simulink model "untitled"  (R2019a)
settings: Solver=ode4  StartTime=0.0  StopTime=100  FixedStep=0.0001  RelTol=1e-3
settings Model: Creator=bahaa  LastModifiedBy=bahaa

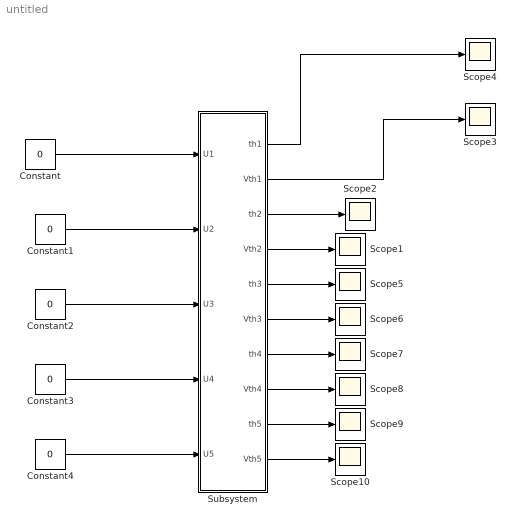
== system untitled ==
  Constant{,1..4} (5 alike) : Constant  Value=0
  Scope{1..10} (10 alike) : Scope
  Subsystem : Subsystem
  wires:
  Constant1/1 -> Subsystem/2(U2)
  Subsystem/4(Vth2) -> Scope1/1
  Constant/1 -> Subsystem/1(U1)
  Constant2/1 -> Subsystem/3(U3)
  Constant3/1 -> Subsystem/4(U4)
  Constant4/1 -> Subsystem/5(U5)
  Subsystem/3(th2) -> Scope2/1
  Subsystem/2(Vth1) -> Scope3/1
  Subsystem/1(th1) -> Scope4/1
  Subsystem/5(th3) -> Scope5/1
  Subsystem/6(Vth3) -> Scope6/1
  Subsystem/7(th4) -> Scope7/1
  Subsystem/8(Vth4) -> Scope8/1
  Subsystem/9(th5) -> Scope9/1
  Subsystem/10(Vth5) -> Scope10/1

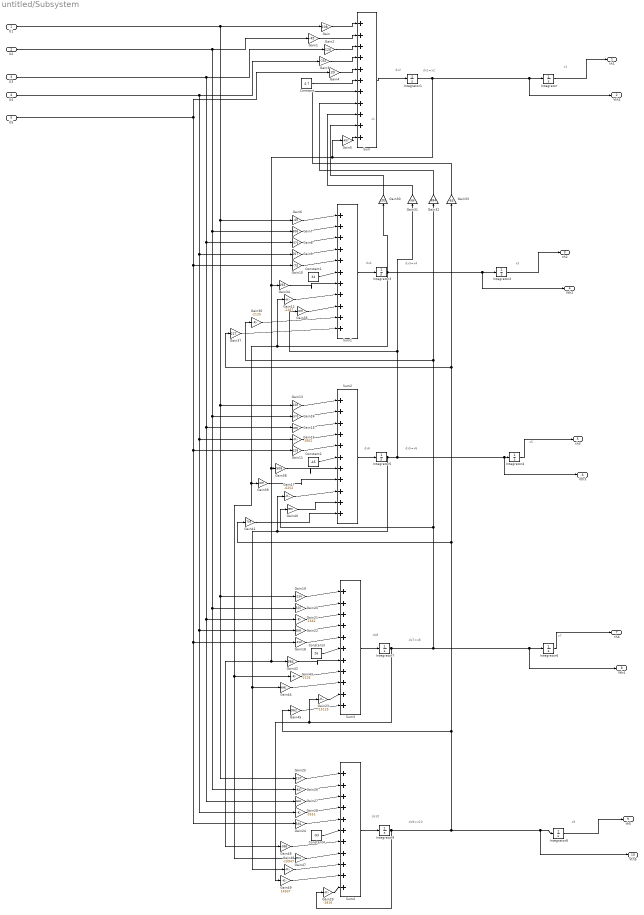
== system untitled/Subsystem ==
  note: dx1=x2
  note: x1
  note: dx2
  note: x3
  note: dx3=x4
  note: x1
  note: x5
  note: dx5=x6
  note: dx7=x8
  note: x7
  note: dx9=x10
  note: x9
  note: dx4
  note: dx6
  note: dx8
  note: dx10
  U1 : Inport
  U2 : Inport  Port=2
  U3 : Inport  Port=3
  U4 : Inport  Port=4
  U5 : Inport  Port=5
  Constant : Constant  Value=4.7
  Constant1 : Constant  Value=34
  Constant2 : Constant  Value=-45
  Constant3 : Constant  Value=26
  Constant4 : Constant  Value=-93
  Gain : Gain  Gain=108
  Gain1 : Gain  Gain=-45
  Gain10 : Gain  Gain=-73
  Gain11 : Gain  Gain=229
  Gain12 : Gain  Gain=-1287
  Gain13 : Gain  Gain=120
  Gain14 : Gain  Gain=-570
  Gain15 : Gain  Gain=1486
  Gain16 : Gain  Gain=-1662
  Gain17 : Gain  Gain=-6252
  Gain18 : Gain  Gain=-313
  Gain19 : Gain  Gain=-234
  Gain2 : Gain  Gain=120
  Gain20 : Gain  Gain=507
  Gain21 : Gain  Gain=-1662
  Gain22 : Gain  Gain=3595
  Gain23 : Gain  Gain=-15125
  Gain24 : Gain  Gain=591
  Gain25 : Gain  Gain=237
  Gain26 : Gain  Gain=-837
  Gain27 : Gain  Gain=2602
  Gain28 : Gain  Gain=-3551
  Gain29 : Gain  Gain=-1816
  Gain3 : Gain  Gain=-234
  Gain30 : Gain  Gain=192
  Gain31 : Gain  Gain=-506
  Gain32 : Gain  Gain=984
  Gain33 : Gain  Gain=-64
  Gain34 : Gain  Gain=192
  Gain35 : Gain  Gain=2400
  Gain36 : Gain  Gain=-2135
  Gain37 : Gain  Gain=227
  Gain38 : Gain  Gain=506
  Gain39 : Gain  Gain=2400
  Gain4 : Gain  Gain=20
  Gain40 : Gain  Gain=6992
  Gain41 : Gain  Gain=-705
  Gain42 : Gain  Gain=984
  Gain43 : Gain  Gain=-2135
  Gain44 : Gain  Gain=6992
  Gain45 : Gain  Gain=962
  Gain46 : Gain  Gain=-998
  Gain47 : Gain  Gain=3521
  Gain48 : Gain  Gain=-10947
  Gain49 : Gain  Gain=14937
  Gain5 : Gain  Gain=-457
  Gain6 : Gain  Gain=-45
  Gain7 : Gain  Gain=306
  Gain8 : Gain  Gain=-570
  Gain9 : Gain  Gain=507
  Integrator{,1..9} (10 alike) : Integrator
  Sum{,1..4} (5 alike) : Sum  Inputs=|+++++++++++
  th1 : Outport
  Vth1 : Outport  Port=2
  th2 : Outport  Port=3
  Vth2 : Outport  Port=4
  th3 : Outport  Port=5
  Vth3 : Outport  Port=6
  th4 : Outport  Port=7
  Vth4 : Outport  Port=8
  th5 : Outport  Port=9
  Vth5 : Outport  Port=10
  wires:
  Sum2/1 -> Integrator5/1
  Gain7/1 -> Sum1/2
  Integrator7/1 -> Gain23/1, Gain49/1, Gain40/1, Gain32/1, Gain36/1, Vth4/1, Integrator6/1
  Sum1/1 -> Integrator3/1
  Gain47/1 -> Sum4/8
  Gain12/1 -> Sum1/8
  Gain9/1 -> Sum1/4
  Gain22/1 -> Sum3/4
  Gain30/1 -> Sum/10
  Gain42/1 -> Sum3/7
  Integrator1/1 -> Vth1/1, Integrator/1, Gain46/1, Gain42/1, Gain38/1, Gain34/1, Gain5/1
  Integrator3/1 -> Gain30/1, Vth2/1, Integrator2/1, Gain47/1, Gain43/1, Gain39/1, Gain12/1
  Gain3/1 -> Sum/4
  Gain13/1 -> Sum2/1
  U1/1 -> Gain25/1, Gain19/1, Gain13/1, Gain6/1, Gain/1
  Sum4/1 -> Integrator9/1
  Gain46/1 -> Sum4/7
  Integrator5/1 -> Gain48/1, Gain44/1, Gain17/1, Gain35/1, Gain31/1, Vth3/1, Integrator4/1
  Gain18/1 -> Sum3/5
  Gain43/1 -> Sum3/8
  Gain31/1 -> Sum/9
  Gain38/1 -> Sum2/7
  U3/1 -> Gain27/1, Gain21/1, Gain15/1, Gain8/1, Gain2/1
  Gain16/1 -> Sum2/4
  Constant1/1 -> Sum1/6
  U2/1 -> Gain26/1, Gain20/1, Gain14/1, Gain7/1, Gain1/1
  Gain33/1 -> Sum/7
  Gain21/1 -> Sum3/3
  Gain39/1 -> Sum2/8
  Constant4/1 -> Sum4/6
  Constant3/1 -> Sum3/6
  Gain1/1 -> Sum/2
  Gain/1 -> Sum/1
  Gain44/1 -> Sum3/9
  Gain17/1 -> Sum2/9
  Gain20/1 -> Sum3/2
  Gain6/1 -> Sum1/1
  Sum3/1 -> Integrator7/1
  Gain19/1 -> Sum3/1
  Gain49/1 -> Sum4/10
  U4/1 -> Gain28/1, Gain22/1, Gain16/1, Gain9/1, Gain3/1
  Integrator8/1 -> th5/1
  U5/1 -> Gain4/1, Gain24/1, Gain18/1, Gain11/1, Gain10/1
  Gain45/1 -> Sum3/11
  Integrator2/1 -> th2/1
  Gain23/1 -> Sum3/10
  Gain29/1 -> Sum4/11
  Constant/1 -> Sum/6
  Gain40/1 -> Sum2/10
  Gain36/1 -> Sum1/10
  Gain34/1 -> Sum1/7
  Integrator9/1 -> Gain29/1, Gain45/1, Gain41/1, Gain37/1, Gain33/1, Vth5/1, Integrator8/1
  Integrator4/1 -> th3/1
  Gain28/1 -> Sum4/4
  Gain27/1 -> Sum4/3
  Gain24/1 -> Sum4/5
  Gain26/1 -> Sum4/2
  Gain25/1 -> Sum4/1
  Gain35/1 -> Sum1/9
  Gain48/1 -> Sum4/9
  Gain32/1 -> Sum/8
  Gain37/1 -> Sum1/11
  Gain41/1 -> Sum2/11
  Gain10/1 -> Sum1/5
  Gain8/1 -> Sum1/3
  Gain2/1 -> Sum/3
  Sum/1 -> Integrator1/1
  Gain5/1 -> Sum/11
  Gain4/1 -> Sum/5
  Gain11/1 -> Sum2/5
  Gain14/1 -> Sum2/2
  Gain15/1 -> Sum2/3
  Constant2/1 -> Sum2/6
  Integrator/1 -> th1/1
  Integrator6/1 -> th4/1
